simulink model "lab2_circuit_model"  (R2025b)
settings: Solver=ode45  StartTime=0.0  StopTime=400  MaxStep=0.5  RelTol=1e-3
undefined symbols (not defined in the file): A, g_f1, g_p2, g_r1, ks, r_m, tau, Vhover, Vlev_out, Voff1, Voff2, Vrail
settings Model: Creator=MTMTAD006  LastModifiedBy=MTMTAD006

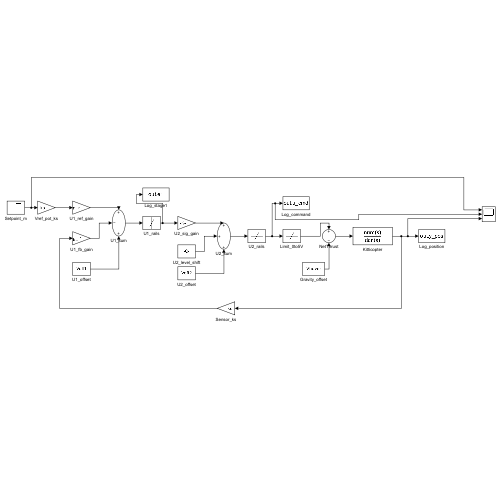
[thumbnail: Simulink's stored preview of the top-level diagram]
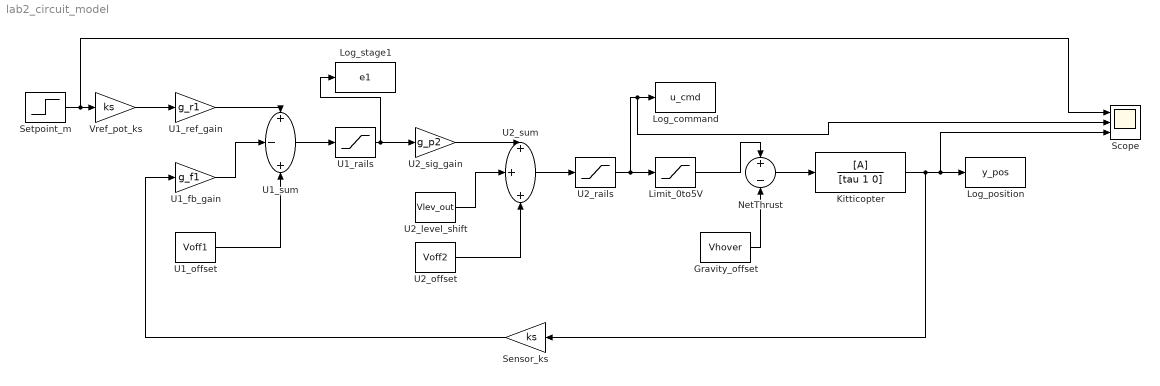
== system lab2_circuit_model ==
  Gravity_offset : Constant  Value=Vhover
  Kitticopter : TransferFcn  Numerator=[A]  Denominator=[tau 1 0]
  Limit_0to5V : Saturate  UpperLimit=5  LowerLimit=0
  Log_command : ToWorkspace  VariableName=u_cmd  SaveFormat=Timeseries  SampleTime=-1
  Log_position : ToWorkspace  VariableName=y_pos  SaveFormat=Timeseries  SampleTime=-1
  Log_stage1 : ToWorkspace  VariableName=e1  SaveFormat=Timeseries  SampleTime=-1
  NetThrust : Sum  Inputs=+-
  Scope : Scope  NumInputPorts=3
      settings: ActiveDisplayYMinimum=-0.77626109939652788  ActiveDisplayYMaximum=6.986349894568753
  Sensor_ks : Gain  Gain=ks
  Setpoint_m : Step  Time=0  After=r_m  SampleTime=0
  U1_fb_gain : Gain  Gain=g_f1
  U1_offset : Constant  Value=Voff1
  U1_rails : Saturate  UpperLimit=Vrail  LowerLimit=-Vrail
  U1_ref_gain : Gain  Gain=g_r1
  U1_sum : Sum  Inputs=+-+
  U2_level_shift : Constant  Value=Vlev_out
  U2_offset : Constant  Value=Voff2
  U2_rails : Saturate  UpperLimit=Vrail  LowerLimit=-Vrail
  U2_sig_gain : Gain  Gain=g_p2
  U2_sum : Sum  Inputs=+++
  Vref_pot_ks : Gain  Gain=ks
  wires:
  Setpoint_m/1 -> Scope/1, Vref_pot_ks/1
  Vref_pot_ks/1 -> U1_ref_gain/1
  U1_ref_gain/1 -> U1_sum/1
  Sensor_ks/1 -> U1_fb_gain/1
  U1_fb_gain/1 -> U1_sum/2
  U1_offset/1 -> U1_sum/3
  U1_sum/1 -> U1_rails/1
  U1_rails/1 -> Log_stage1/1, U2_sig_gain/1
  U2_sig_gain/1 -> U2_sum/1
  U2_level_shift/1 -> U2_sum/2
  U2_offset/1 -> U2_sum/3
  U2_sum/1 -> U2_rails/1
  U2_rails/1 -> Scope/2, Log_command/1, Limit_0to5V/1
  Limit_0to5V/1 -> NetThrust/1
  Gravity_offset/1 -> NetThrust/2
  NetThrust/1 -> Kitticopter/1
  Kitticopter/1 -> Scope/3, Log_position/1, Sensor_ks/1
